simulink model "task4_Kpop"  (R2023a)
settings: Solver=ode45  StartTime=0  StopTime=1200  RelTol=1e-6  AbsTol=1e-9
InitFcn:
  | Pi=10; beta=8.3e-4; mu=1/144; b=1/24; eps=0.75; P=2; N=1; S0=1500; B0=3; R0=0;
Description:
  | Zadanie 4 (2.27): S,B,R=u[1..3]; P,N-doli pozitivnyh i negativnyh SMI.
settings Model: Creator=maybn  LastModifiedBy=maybn
settings OptimizationCC: BlockReduction=off  BooleanDataType=off
settings DebuggingCC: SaveWithParameterizedLinksMsg=none  UnderspecifiedInitializationDetection=Classic  MergeDetectMultiDrivingBlocksExec=none  SignalResolutionControl=TryResolveAllWithWarning
settings HardwareCC: TargetUnknown=on
settings ModelReferenceCC: PropagateSignalLabelsOutOfModel=off

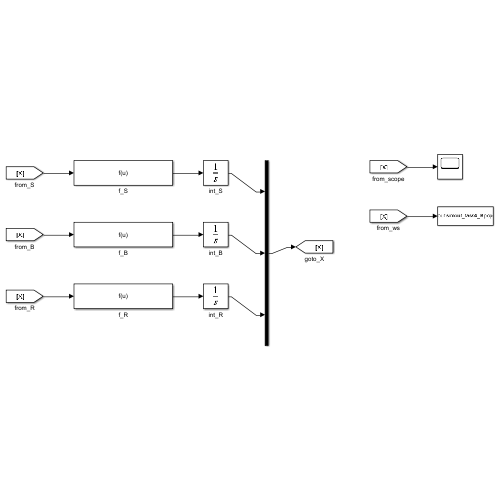
[thumbnail: Simulink's stored preview of the top-level diagram]
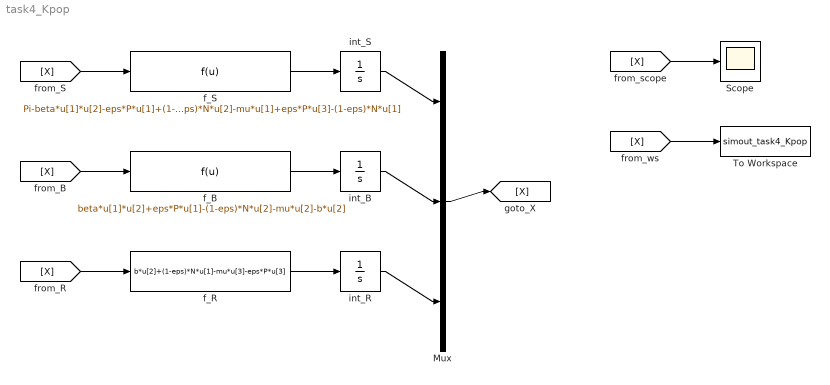
== system task4_Kpop ==
  Mux : Mux  Inputs=3
  Scope : Scope
  To Workspace : ToWorkspace  VariableName=simout_task4_Kpop
  f_B : Fcn  Expr=beta*u[1]*u[2]+eps*P*u[1]-(1-eps)*N*u[2]-mu*u[2]-b*u[2]
  f_R : Fcn  Expr=b*u[2]+(1-eps)*N*u[1]-mu*u[3]-eps*P*u[3]
  f_S : Fcn  Expr=Pi-beta*u[1]*u[2]-eps*P*u[1]+(1-eps)*N*u[2]-mu*u[1]+eps*P*u[3]-(1-eps)*N*u[1]
  int_B : Integrator  InitialCondition=B0
  int_R : Integrator  InitialCondition=R0
  int_S : Integrator  InitialCondition=S0
  wires:
  [X] -> f_S/1
  f_S/1 -> int_S/1
  int_S/1 -> Mux/1
  [X] -> f_B/1
  f_B/1 -> int_B/1
  int_B/1 -> Mux/2
  [X] -> f_R/1
  f_R/1 -> int_R/1
  int_R/1 -> Mux/3
  Mux/1 -> [X]
  [X] -> Scope/1
  [X] -> To Workspace/1
